simulink library "sm_wheel_loader_lib"  (R2025a)
settings: Solver=VariableStepAuto  StartTime=0.0  StopTime=10.0  RelTol=1e-3
undefined symbols (not defined in the file): AToTOrificeVector, BiPOrificeVector, boomHEArea, boomREArea, BToTOrificeVector, fluids, GRake, GToothL, GToothR, HMPST, HydFcnParams, logLoad, Position, PToAOrificeVector, PToBOrificeVector, RakeL, RakeR, testInput, Wheel_Loader, X, Y, Z
libraries: sm_lib x694, fl_lib x183, nesl_utility x74, SimscapeFluids_lib x62, sdl_lib x25, cvt_components_lib x25, simulink_extras x5, $bdroot x4, wheel_loader_contact_lib x4, ee_lib x2, SignalEditorBlockLib x1, batteryecm_lib x1
(part 5 of 26)

== system sm_wheel_loader_lib/CVT Power Split Hydromechanical/Hydrostatic/Motor Leakage ==
  Case Drain : fl_lib/Isothermal Liquid/Elements/Reservoir (IL)  reservoir_type=foundation.enum.constant_controlled.constant  pressure_spec=foundation.enum.pressure_spec.atmospheric  reservoir_pressure=0.101325 MPa
  Leakage A : fl_lib/Isothermal Liquid/Elements/Laminar Leakage (IL)  cross_section_geometry=foundation.enum.cross_section_geometry.custom  diameter=1e-3 m  inner_diameter=5e-4 m  outer_diameter=1e-3 m  width=1e-3 m  height=0.1 m  major_axis=1e-3 m  minor_axis=5e-4 m  side_length=1e-3 m  length=5 m  resistance=1e7 s*MPa/m^3
      settings: InternalSimscapePortConfiguration="{\"Bottom\":[],\"Left\":[{\"id\":\"A\",\"label\":\"A\",\"type\":\"foundation.isothermal_liquid.isothermal_liquid\"}],\"Right\":[{\"id\":\"B\",\"label\":\"B\",\"type\":\"foundation.isothermal_liquid.isothermal_liquid\"}],\"Top\":[]}"
  Leakage B : fl_lib/Isothermal Liquid/Elements/Laminar Leakage (IL)  cross_section_geometry=foundation.enum.cross_section_geometry.custom  diameter=1e-3 m  inner_diameter=5e-4 m  outer_diameter=1e-3 m  width=1e-3 m  height=0.1 m  major_axis=1e-3 m  minor_axis=5e-4 m  side_length=1e-3 m  length=5 m  resistance=1e7 s*MPa/m^3
      settings: InternalSimscapePortConfiguration="{\"Bottom\":[],\"Left\":[{\"id\":\"A\",\"label\":\"A\",\"type\":\"foundation.isothermal_liquid.isothermal_liquid\"}],\"Right\":[{\"id\":\"B\",\"label\":\"B\",\"type\":\"foundation.isothermal_liquid.isothermal_liquid\"}],\"Top\":[]}"
  A : PMIOPort  Side=Left
  B : PMIOPort  Port=2  Side=Left
  connections:
  Leakage A/LConn1 -- A/RConn1
  Leakage B/RConn1 -- Case Drain/LConn1 -- Leakage A/RConn1
  Leakage B/LConn1 -- B/RConn1

== system sm_wheel_loader_lib/CVT Power Split Hydromechanical/Hydrostatic/Pump Leakage ==
  Case Drain : fl_lib/Isothermal Liquid/Elements/Reservoir (IL)  reservoir_type=foundation.enum.constant_controlled.constant  pressure_spec=foundation.enum.pressure_spec.atmospheric  reservoir_pressure=0.101325 MPa
  Leakage A : fl_lib/Isothermal Liquid/Elements/Laminar Leakage (IL)  cross_section_geometry=foundation.enum.cross_section_geometry.custom  diameter=1e-3 m  inner_diameter=5e-4 m  outer_diameter=1e-3 m  width=1e-3 m  height=0.1 m  major_axis=1e-3 m  minor_axis=5e-4 m  side_length=1e-3 m  length=5 m  resistance=1e7 s*MPa/m^3
      settings: InternalSimscapePortConfiguration="{\"Bottom\":[],\"Left\":[{\"id\":\"A\",\"label\":\"A\",\"type\":\"foundation.isothermal_liquid.isothermal_liquid\"}],\"Right\":[{\"id\":\"B\",\"label\":\"B\",\"type\":\"foundation.isothermal_liquid.isothermal_liquid\"}],\"Top\":[]}"
  Leakage B : fl_lib/Isothermal Liquid/Elements/Laminar Leakage (IL)  cross_section_geometry=foundation.enum.cross_section_geometry.custom  diameter=1e-3 m  inner_diameter=5e-4 m  outer_diameter=1e-3 m  width=1e-3 m  height=0.1 m  major_axis=1e-3 m  minor_axis=5e-4 m  side_length=1e-3 m  length=5 m  resistance=1e7 s*MPa/m^3
      settings: InternalSimscapePortConfiguration="{\"Bottom\":[],\"Left\":[{\"id\":\"A\",\"label\":\"A\",\"type\":\"foundation.isothermal_liquid.isothermal_liquid\"}],\"Right\":[{\"id\":\"B\",\"label\":\"B\",\"type\":\"foundation.isothermal_liquid.isothermal_liquid\"}],\"Top\":[]}"
  B : PMIOPort  Side=Left
  A : PMIOPort  Port=2  Side=Left
  connections:
  Leakage A/LConn1 -- A/RConn1
  Leakage B/RConn1 -- Leakage A/RConn1 -- Case Drain/LConn1
  Leakage B/LConn1 -- B/RConn1

== system sm_wheel_loader_lib/Controller/CVT Ratio Ctrl/Range Calculation ==
  Ratio (-) : Inport
  Check Range 0 or higher : Switch  Threshold=XY_I(1,2)  SaturateOnIntegerOverflow=off  InputSameDT=off
  Check Range 2 or higher : Switch  Threshold=XY_I(2,2)  SaturateOnIntegerOverflow=off  InputSameDT=off
  Check Range 3 or higher : Switch  Threshold=XY_I(3,2)  SaturateOnIntegerOverflow=off  InputSameDT=off
  Check Range 4 : Switch  Threshold=XY_I(4,2)  SaturateOnIntegerOverflow=off  InputSameDT=off
  Constant1 : Constant  Value=2  SampleTime=HMPST.Simu.TimeStep
  Constant2 : Constant  SampleTime=HMPST.Simu.TimeStep
  Constant3 : Constant  Value=-1  SampleTime=HMPST.Simu.TimeStep
  Constant4 : Constant  Value=3  SampleTime=HMPST.Simu.TimeStep
  Constant5 : Constant  Value=4  SampleTime=HMPST.Simu.TimeStep
  Range (-) : Outport
  wires:
  Check Range 2 or higher/1 -> Check Range 0 or higher/1
  Constant2/1 -> Check Range 2 or higher/3
  Constant3/1 -> Check Range 0 or higher/3
  Check Range 0 or higher/1 -> Range (-)/1  "Range"
  Check Range 3 or higher/1 -> Check Range 2 or higher/1
  Constant1/1 -> Check Range 3 or higher/3
  Check Range 4/1 -> Check Range 3 or higher/1
  Constant4/1 -> Check Range 4/3
  Constant5/1 -> Check Range 4/1
  Ratio (-)/1 -> Check Range 2 or higher/2, Check Range 3 or higher/2, Check Range 4/2, Check Range 0 or higher/2

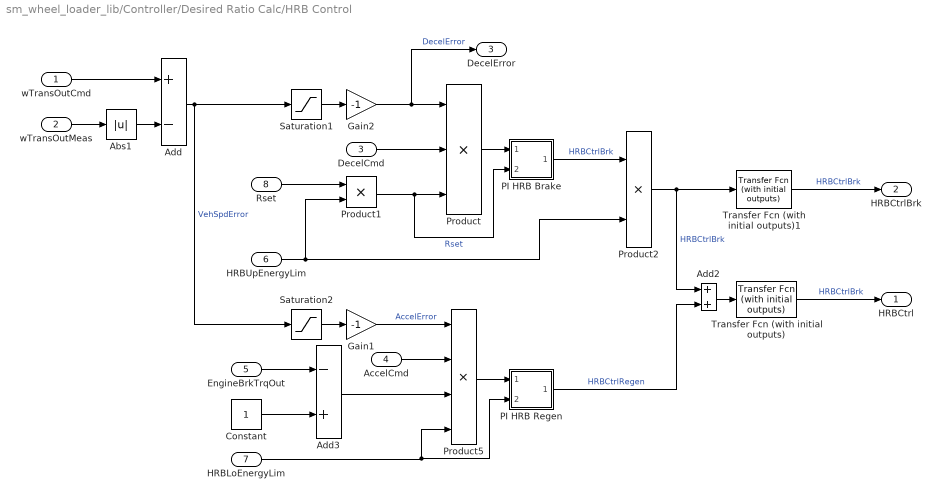
== system sm_wheel_loader_lib/Controller/Desired Ratio Calc/HRB Control ==
  wTransOutCmd : Inport
  wTransOutMeas : Inport  Port=2
  DecelCmd : Inport  Port=3
  AccelCmd : Inport  Port=4
  EngineBrkTrqOut : Inport  Port=5
  HRBUpEnergyLim : Inport  Port=6
  HRBLoEnergyLim : Inport  Port=7
  Rset : Inport  Port=8
  Abs1 : Abs  ZeroCross=off  SaturateOnIntegerOverflow=off
  Add : Sum  Inputs=+-
  Add2 : Sum
  Add3 : Sum  Inputs=-+
  Constant : Constant
  Gain1 : Gain  Gain=-1
  Gain2 : Gain  Gain=-1
  PI HRB Brake : Subsystem
  PI HRB Regen : Subsystem
  Product : Product  Inputs=3
  Product1 : Product
  Product2 : Product
  Product5 : Product  Inputs=4
  Saturation1 : Saturate  UpperLimit=0  LowerLimit=-inf  ZeroCross=off
  Saturation2 : Saturate  UpperLimit=inf  LowerLimit=0  ZeroCross=off
  Transfer Fcn (with initial outputs) : simulink_extras/Additional Linear/Transfer Fcn (with initial outputs)  N=[0.01]  D=[0.05 1]  Y0=0  U0=0
  Transfer Fcn (with initial outputs)1 : simulink_extras/Additional Linear/Transfer Fcn (with initial outputs)  N=[0.01]  D=[0.05 1]  Y0=0  U0=0
  HRBCtrl : Outport
  HRBCtrlBrk : Outport  Port=2
  DecelError : Outport  Port=3
  wires:
  Product/1 -> PI HRB Brake/1(error)
  Product5/1 -> PI HRB Regen/1(error)
  Gain1/1 -> Product5/1  "AccelError"
  Transfer Fcn (with initial outputs)1/1 -> HRBCtrlBrk/1  "HRBCtrlBrk"
  Rset/1 -> Product1/1
  EngineBrkTrqOut/1 -> Add3/1
  wTransOutCmd/1 -> Add/1
  PI HRB Brake/1(ctrl) -> Product2/1  "HRBCtrlBrk"
  wTransOutMeas/1 -> Abs1/1
  Gain2/1 -> Product/1, DecelError/1  "DecelError"
  AccelCmd/1 -> Product5/2
  Saturation1/1 -> Gain2/1
  Saturation2/1 -> Gain1/1
  PI HRB Regen/1(ctrl) -> Add2/2  "HRBCtrlRegen"
  HRBUpEnergyLim/1 -> Product1/2, Product2/2
  Abs1/1 -> Add/2
  DecelCmd/1 -> Product/2
  Product2/1 -> Transfer Fcn (with initial outputs)1/1, Add2/1  "HRBCtrlBrk"
  Add/1 -> Saturation1/1, Saturation2/1  "VehSpdError"
  Transfer Fcn (with initial outputs)/1 -> HRBCtrl/1  "HRBCtrlBrk"
  Constant/1 -> Add3/2
  Product1/1 -> Product/3, PI HRB Brake/2(Rset)  "Rset"
  Add3/1 -> Product5/3
  HRBLoEnergyLim/1 -> Product5/4, PI HRB Regen/2(Rset)
  Add2/1 -> Transfer Fcn (with initial outputs)/1

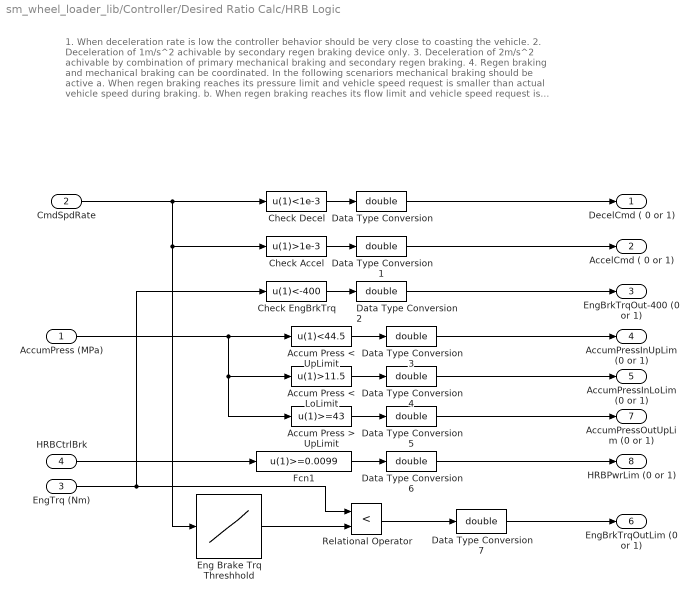
== system sm_wheel_loader_lib/Controller/Desired Ratio Calc/HRB Logic ==
  note: 1. When deceleration rate is low the controller behavior should be very close to coasting the vehicle.
      | 2. Deceleration of 1m/s^2 achivable by secondary regen braking device only.
      | 3. Deceleration of 2m/s^2 achivable by combination of primary mechanical braking and secondary regen braking.
      | 4. Regen braking and mechanical braking can be coordinated. In the following scenariors mechanical braking should be active
      | a. When regen braking reaches its pressure limit and vehicle speed request is smaller than actual vehicle speed during braking.
      | b. When regen braking reaches its flow limit and vehicle speed request is smaller than actual vehicle speed during braking.
      | 5. Energy in the accumulator will be released when accelerating and the accumulator pressure is above minimum working pressure.
      | Energy release rate should not cause engine over speeding.
      | 6. If engine over speed limit is reached disengage master clutch/shut down the engine.
  AccumPress (MPa) : Inport
  CmdSpdRate : Inport  Port=2
  EngTrq (Nm) : Inport  Port=3
  HRBCtrlBrk : Inport  Port=4
  Accum Press < LoLimit : Fcn  Expr=u(1)>11.5
  Accum Press < UpLimit : Fcn  Expr=u(1)<44.5
  Accum Press > UpLimit : Fcn  Expr=u(1)>=43
  Check Accel : Fcn  Expr=u(1)>1e-3
  Check Decel : Fcn  Expr=u(1)<1e-3
  Check EngBrkTrq : Fcn  Expr=u(1)<-400
  Data Type Conversion{,1..7} (8 alike) : DataTypeConversion  OutDataTypeStr=double  SaturateOnIntegerOverflow=off  RndMeth=Floor
  Eng Brake Trq Threshhold : Lookup_n-D  NumberOfTableDimensions=1  BreakpointsForDimension1=[-3 -2 -1 -0.5 0 1]  Table=[-450 -450 -225 -113 0 0]*0.6  InternalRulePriority=Speed  RndMeth=Simplest
  Fcn1 : Fcn  Expr=u(1)>=0.0099
  Relational Operator : RelationalOperator  Operator=<  OutDataTypeStr=boolean  ZeroCross=off  InputSameDT=off
  DecelCmd ( 0 or 1) : Outport
  AccelCmd ( 0 or 1) : Outport  Port=2
  EngBrkTrqOut-400 (0 or 1) : Outport  Port=3
  AccumPressInUpLim (0 or 1) : Outport  Port=4
  AccumPressInLoLim (0 or 1) : Outport  Port=5
  EngBrkTrqOutLim (0 or 1) : Outport  Port=6
  AccumPressOutUpLim (0 or 1) : Outport  Port=7
  HRBPwrLim (0 or 1) : Outport  Port=8
  wires:
  Check Decel/1 -> Data Type Conversion/1
  Data Type Conversion/1 -> DecelCmd ( 0 or 1)/1
  EngTrq (Nm)/1 -> Relational Operator/1, Check EngBrkTrq/1
  CmdSpdRate/1 -> Check Decel/1, Eng Brake Trq Threshhold/1, Check Accel/1
  Eng Brake Trq Threshhold/1 -> Relational Operator/2
  AccumPress (MPa)/1 -> Accum Press < LoLimit/1, Accum Press > UpLimit/1, Accum Press < UpLimit/1
  Accum Press < UpLimit/1 -> Data Type Conversion3/1
  Relational Operator/1 -> Data Type Conversion7/1
  Accum Press > UpLimit/1 -> Data Type Conversion5/1
  HRBCtrlBrk/1 -> Fcn1/1
  Fcn1/1 -> Data Type Conversion6/1
  Accum Press < LoLimit/1 -> Data Type Conversion4/1
  Check Accel/1 -> Data Type Conversion1/1
  Check EngBrkTrq/1 -> Data Type Conversion2/1
  Data Type Conversion1/1 -> AccelCmd ( 0 or 1)/1
  Data Type Conversion2/1 -> EngBrkTrqOut-400 (0 or 1)/1
  Data Type Conversion3/1 -> AccumPressInUpLim (0 or 1)/1
  Data Type Conversion4/1 -> AccumPressInLoLim (0 or 1)/1
  Data Type Conversion5/1 -> AccumPressOutUpLim (0 or 1)/1
  Data Type Conversion6/1 -> HRBPwrLim (0 or 1)/1
  Data Type Conversion7/1 -> EngBrkTrqOutLim (0 or 1)/1

== system sm_wheel_loader_lib/Controller/Desired Ratio Calc/MB Control ==
  Decel Error : Inport
  wTransOutCmd : Inport  Port=2
  Rset : Inport  Port=3
  AccumLimUp : Inport  Port=4
  HRBPowerLim : Inport  Port=5
  Add1 : Sum  Inputs=+++
  Compare To Constant : simulink/Logic and Bit Operations/Compare To Constant  relop=<=  const=0.02  OutDataTypeStr=boolean
  Data Type Conversion : DataTypeConversion  OutDataTypeStr=double  SaturateOnIntegerOverflow=off  RndMeth=Floor
  PI MB No HRB : Subsystem
  PI MB with MRB : Subsystem
  Product3 : Product  Inputs=3
  Product4 : Product
  Out1 : Outport
  wires:
  HRBPowerLim/1 -> Product4/2
  AccumLimUp/1 -> Product3/3
  wTransOutCmd/1 -> Compare To Constant/1
  PI MB with MRB/1(ctrl) -> Add1/3
  Add1/1 -> Out1/1
  Product4/1 -> PI MB with MRB/1(error)
  PI MB No HRB/1(ctrl) -> Add1/2
  Data Type Conversion/1 -> Add1/1
  Compare To Constant/1 -> Data Type Conversion/1
  Rset/1 -> PI MB with MRB/2(Rset), PI MB No HRB/2(Rset), Product3/2
  Product3/1 -> PI MB No HRB/1(error)
  Decel Error/1 -> Product4/1, Product3/1

== system sm_wheel_loader_lib/Controller/Desired Ratio Calc/VehSpdDir ==
  u : Inport
  Constant1 : Constant
  Constant2 : Constant  Value=-1
  Constant3 : Constant  Value=0
  Gain : Gain  Gain=-1
  Switch : Switch  Criteria=u2 > Threshold  Threshold=0.001  SaturateOnIntegerOverflow=off  InputSameDT=off
  Switch1 : Switch  Criteria=u2 > Threshold  Threshold=0.001  SaturateOnIntegerOverflow=off  InputSameDT=off
  u_dir : Outport
  wires:
  Gain/1 -> Switch1/2
  Switch/1 -> u_dir/1
  u/1 -> Switch/2, Gain/1
  Constant1/1 -> Switch/1
  Switch1/1 -> Switch/3
  Constant3/1 -> Switch1/3
  Constant2/1 -> Switch1/1

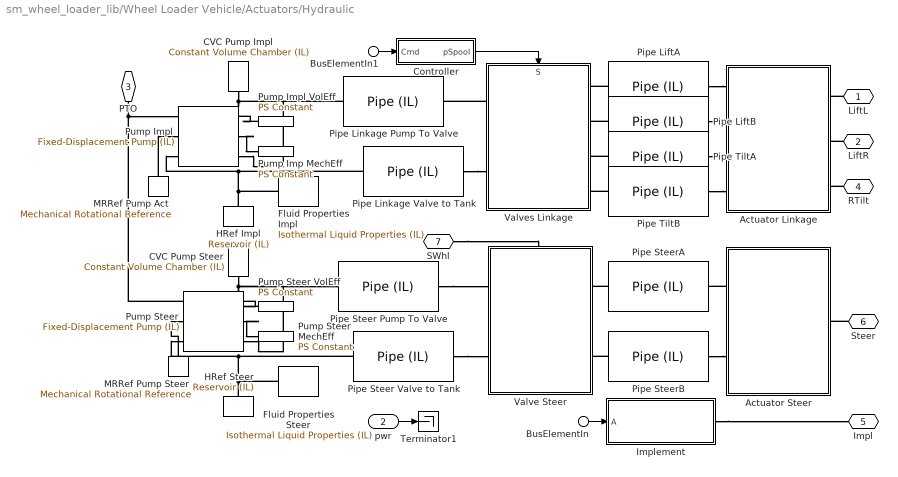
== system sm_wheel_loader_lib/Wheel Loader Vehicle/Actuators/Hydraulic ==
  BusElementIn : Inport  PortName=Cmd  Element=Actuator
  BusElementIn1 : Inport  PortName=Cmd  Element=Operator
  pwr : Inport  Port=2
  Actuator Linkage : Subsystem
      mask Display: image('sm_wheel_loader_actuator_linkage_IMAGE.png');
  Actuator Steer : Subsystem
      mask Display: image('sm_wheel_loader_actuator_steer_IMAGE.png');
  CVC Pump Impl : fl_lib/Isothermal Liquid/Elements/Constant Volume Chamber (IL)  volume=HydFcnParams.pump.chamberVol mm^3  p_I_specify=off  p_I_priority=High  p_I=0.101325 MPa  p_I_nominal_specify=off  p_I_nominal_value=1  p_I_nominal_unit=MPa
      settings: InternalSimscapePortConfiguration="{\"Bottom\":[],\"Left\":[{\"id\":\"A\",\"label\":\"A\",\"type\":\"foundation.isothermal_liquid.isothermal_liquid\"}],\"Right\":[],\"Top\":[]}"
  CVC Pump Steer : fl_lib/Isothermal Liquid/Elements/Constant Volume Chamber (IL)  volume=HydFcnParams.steerPump.chamberVol mm^3  p_I_specify=off  p_I_priority=High  p_I=0.101325 MPa  p_I_nominal_specify=off  p_I_nominal_value=1  p_I_nominal_unit=MPa
      settings: InternalSimscapePortConfiguration="{\"Bottom\":[],\"Left\":[{\"id\":\"A\",\"label\":\"A\",\"type\":\"foundation.isothermal_liquid.isothermal_liquid\"}],\"Right\":[],\"Top\":[]}"
  Controller : Subsystem
  Fluid Properties Impl : fl_lib/Isothermal Liquid/Utilities/Isothermal Liquid Properties (IL)  rho_L_atm=870 kg/m^3  bulk_modulus_model=foundation.enum.bulk_modulus_model.const  beta_gain=6  beta_L_atm=1.45e9 Pa  nu_atm=46 mm^2/s  p_atm=0.101325 MPa  p_min=0.1 Pa  properties_range_check=simscape.enum.assert.action.error  air_fraction=0.005  polytropic_index=1.0  rho_g_atm=1.225 kg/m^3  air_dissolution_model=simscape.enum.onoff.off  p_crit=3 MPa
  Fluid Properties Steer : fl_lib/Isothermal Liquid/Utilities/Isothermal Liquid Properties (IL)  rho_L_atm=870 kg/m^3  bulk_modulus_model=foundation.enum.bulk_modulus_model.const  beta_gain=6  beta_L_atm=1.45e9 Pa  nu_atm=46 mm^2/s  p_atm=0.101325 MPa  p_min=0.1 Pa  properties_range_check=simscape.enum.assert.action.error  air_fraction=0.005  polytropic_index=1.0  rho_g_atm=1.225 kg/m^3  air_dissolution_model=simscape.enum.onoff.off  p_crit=3 MPa
  HRef Impl : fl_lib/Isothermal Liquid/Elements/Reservoir (IL)  reservoir_type=foundation.enum.constant_controlled.constant  pressure_spec=foundation.enum.pressure_spec.atmospheric  reservoir_pressure=0.101325 MPa
  HRef Steer : fl_lib/Isothermal Liquid/Elements/Reservoir (IL)  reservoir_type=foundation.enum.constant_controlled.constant  pressure_spec=foundation.enum.pressure_spec.atmospheric  reservoir_pressure=0.101325 MPa
  Implement : Subsystem  Variant=on  VariantControlMode=label  VariantControl=Grapple Rake  LabelModeActiveChoice=Bucket
      settings: AttributesFormatString=%<LabelModeActiveChoice>
  MRRef Pump Act : fl_lib/Mechanical/Rotational Elements/Mechanical Rotational Reference
  MRRef Pump Steer : fl_lib/Mechanical/Rotational Elements/Mechanical Rotational Reference
  Pipe LiftA : fl_lib/Isothermal Liquid/Elements/Pipe (IL)  length=HydFcnParams.pipes.length mm  area=HydFcnParams.pipe.crossSectArea mm^2  Dh=HydFcnParams.pipes.hydraulicDiam mm  length_add=1 m  roughness=15e-6 m  Re_lam=2000  Re_tur=4000  shape_factor=64  dynamic_compressibility=simscape.enum.onoff.off  inertia=simscape.enum.onoff.off  p0=0.101325 MPa  mdot0=0 kg/s
      settings: InternalSimscapePortConfiguration="{\"Bottom\":[],\"Left\":[{\"id\":\"A\",\"label\":\"A\",\"type\":\"foundation.isothermal_liquid.isothermal_liquid\"}],\"Right\":[{\"id\":\"B\",\"label\":\"B\",\"type\":\"foundation.isothermal_liquid.isothermal_liquid\"}],\"Top\":[]}"
  Pipe LiftB : fl_lib/Isothermal Liquid/Elements/Pipe (IL)  length=HydFcnParams.pipes.length mm  area=HydFcnParams.pipe.crossSectArea mm^2  Dh=HydFcnParams.pipes.hydraulicDiam mm  length_add=1 m  roughness=15e-6 m  Re_lam=2000  Re_tur=4000  shape_factor=64  dynamic_compressibility=simscape.enum.onoff.off  inertia=simscape.enum.onoff.off  p0=0.101325 MPa  mdot0=0 kg/s
      settings: InternalSimscapePortConfiguration="{\"Bottom\":[],\"Left\":[{\"id\":\"A\",\"label\":\"A\",\"type\":\"foundation.isothermal_liquid.isothermal_liquid\"}],\"Right\":[{\"id\":\"B\",\"label\":\"B\",\"type\":\"foundation.isothermal_liquid.isothermal_liquid\"}],\"Top\":[]}"
  Pipe Linkage Pump To Valve : fl_lib/Isothermal Liquid/Elements/Pipe (IL)  length=HydFcnParams.pipes.length mm  area=HydFcnParams.pipe.crossSectArea mm^2  Dh=HydFcnParams.pipes.hydraulicDiam mm  length_add=1 m  roughness=15e-6 m  Re_lam=2000  Re_tur=4000  shape_factor=64  dynamic_compressibility=simscape.enum.onoff.off  inertia=simscape.enum.onoff.off  p0=0.101325 MPa  mdot0=0 kg/s
      settings: InternalSimscapePortConfiguration="{\"Bottom\":[],\"Left\":[{\"id\":\"A\",\"label\":\"A\",\"type\":\"foundation.isothermal_liquid.isothermal_liquid\"}],\"Right\":[{\"id\":\"B\",\"label\":\"B\",\"type\":\"foundation.isothermal_liquid.isothermal_liquid\"}],\"Top\":[]}"
  Pipe Linkage Valve to Tank : fl_lib/Isothermal Liquid/Elements/Pipe (IL)  length=HydFcnParams.pipes.length mm  area=HydFcnParams.pipe.crossSectArea mm^2  Dh=HydFcnParams.pipes.hydraulicDiam mm  length_add=1 m  roughness=15e-6 m  Re_lam=2000  Re_tur=4000  shape_factor=64  dynamic_compressibility=simscape.enum.onoff.off  inertia=simscape.enum.onoff.off  p0=0.101325 MPa  mdot0=0 kg/s
      settings: InternalSimscapePortConfiguration="{\"Bottom\":[],\"Left\":[{\"id\":\"A\",\"label\":\"A\",\"type\":\"foundation.isothermal_liquid.isothermal_liquid\"}],\"Right\":[{\"id\":\"B\",\"label\":\"B\",\"type\":\"foundation.isothermal_liquid.isothermal_liquid\"}],\"Top\":[]}"
  Pipe Steer Pump To Valve : fl_lib/Isothermal Liquid/Elements/Pipe (IL)  length=HydFcnParams.pipes.length mm  area=HydFcnParams.pipe.crossSectArea mm^2  Dh=HydFcnParams.pipes.hydraulicDiam mm  length_add=1 m  roughness=15e-6 m  Re_lam=2000  Re_tur=4000  shape_factor=64  dynamic_compressibility=simscape.enum.onoff.off  inertia=simscape.enum.onoff.off  p0=0.101325 MPa  mdot0=0 kg/s
      settings: InternalSimscapePortConfiguration="{\"Bottom\":[],\"Left\":[{\"id\":\"A\",\"label\":\"A\",\"type\":\"foundation.isothermal_liquid.isothermal_liquid\"}],\"Right\":[{\"id\":\"B\",\"label\":\"B\",\"type\":\"foundation.isothermal_liquid.isothermal_liquid\"}],\"Top\":[]}"
  Pipe Steer Valve to Tank : fl_lib/Isothermal Liquid/Elements/Pipe (IL)  length=HydFcnParams.pipes.length mm  area=HydFcnParams.pipe.crossSectArea mm^2  Dh=HydFcnParams.pipes.hydraulicDiam mm  length_add=1 m  roughness=15e-6 m  Re_lam=2000  Re_tur=4000  shape_factor=64  dynamic_compressibility=simscape.enum.onoff.off  inertia=simscape.enum.onoff.off  p0=0.101325 MPa  mdot0=0 kg/s
      settings: InternalSimscapePortConfiguration="{\"Bottom\":[],\"Left\":[{\"id\":\"A\",\"label\":\"A\",\"type\":\"foundation.isothermal_liquid.isothermal_liquid\"}],\"Right\":[{\"id\":\"B\",\"label\":\"B\",\"type\":\"foundation.isothermal_liquid.isothermal_liquid\"}],\"Top\":[]}"
  Pipe SteerA : fl_lib/Isothermal Liquid/Elements/Pipe (IL)  length=HydFcnParams.pipes.length mm  area=HydFcnParams.pipe.crossSectArea mm^2  Dh=HydFcnParams.pipes.hydraulicDiam mm  length_add=1 m  roughness=15e-6 m  Re_lam=2000  Re_tur=4000  shape_factor=64  dynamic_compressibility=simscape.enum.onoff.off  inertia=simscape.enum.onoff.off  p0=0.101325 MPa  mdot0=0 kg/s
      settings: InternalSimscapePortConfiguration="{\"Bottom\":[],\"Left\":[{\"id\":\"A\",\"label\":\"A\",\"type\":\"foundation.isothermal_liquid.isothermal_liquid\"}],\"Right\":[{\"id\":\"B\",\"label\":\"B\",\"type\":\"foundation.isothermal_liquid.isothermal_liquid\"}],\"Top\":[]}"
  Pipe SteerB : fl_lib/Isothermal Liquid/Elements/Pipe (IL)  length=HydFcnParams.pipes.length mm  area=HydFcnParams.pipe.crossSectArea mm^2  Dh=HydFcnParams.pipes.hydraulicDiam mm  length_add=1 m  roughness=15e-6 m  Re_lam=2000  Re_tur=4000  shape_factor=64  dynamic_compressibility=simscape.enum.onoff.off  inertia=simscape.enum.onoff.off  p0=0.101325 MPa  mdot0=0 kg/s
      settings: InternalSimscapePortConfiguration="{\"Bottom\":[],\"Left\":[{\"id\":\"A\",\"label\":\"A\",\"type\":\"foundation.isothermal_liquid.isothermal_liquid\"}],\"Right\":[{\"id\":\"B\",\"label\":\"B\",\"type\":\"foundation.isothermal_liquid.isothermal_liquid\"}],\"Top\":[]}"
  Pipe TiltA : fl_lib/Isothermal Liquid/Elements/Pipe (IL)  length=HydFcnParams.pipes.length mm  area=HydFcnParams.pipe.crossSectArea mm^2  Dh=HydFcnParams.pipes.hydraulicDiam mm  length_add=1 m  roughness=15e-6 m  Re_lam=2000  Re_tur=4000  shape_factor=64  dynamic_compressibility=simscape.enum.onoff.off  inertia=simscape.enum.onoff.off  p0=0.101325 MPa  mdot0=0 kg/s
      settings: InternalSimscapePortConfiguration="{\"Bottom\":[],\"Left\":[{\"id\":\"A\",\"label\":\"A\",\"type\":\"foundation.isothermal_liquid.isothermal_liquid\"}],\"Right\":[{\"id\":\"B\",\"label\":\"B\",\"type\":\"foundation.isothermal_liquid.isothermal_liquid\"}],\"Top\":[]}"
  Pipe TiltB : fl_lib/Isothermal Liquid/Elements/Pipe (IL)  length=HydFcnParams.pipes.length mm  area=HydFcnParams.pipe.crossSectArea mm^2  Dh=HydFcnParams.pipes.hydraulicDiam mm  length_add=1 m  roughness=15e-6 m  Re_lam=2000  Re_tur=4000  shape_factor=64  dynamic_compressibility=simscape.enum.onoff.off  inertia=simscape.enum.onoff.off  p0=0.101325 MPa  mdot0=0 kg/s
      settings: InternalSimscapePortConfiguration="{\"Bottom\":[],\"Left\":[{\"id\":\"A\",\"label\":\"A\",\"type\":\"foundation.isothermal_liquid.isothermal_liquid\"}],\"Right\":[{\"id\":\"B\",\"label\":\"B\",\"type\":\"foundation.isothermal_liquid.isothermal_liquid\"}],\"Top\":[]}"
  Pump Impl : SimscapeFluids_lib/Isothermal Liquid/Pumps & Motors/Fixed-Displacement Pump (IL)  leakage_friction_spec=fluids.isothermal_liquid.pumps_motors.enum.pump_motor_loss_spec.input_efficiency  displacement=HydFcnParams.pump.displacement cm^3/rev  omega_nominal=HydFcnParams.pump.nomSpeed rpm  p_nominal=HydFcnParams.pump.nomPrGain bar  vol_eff_nominal=HydFcnParams.pump.volEff  mech_eff_nominal=HydFcnParams.pump.mechEff  no_load_torque=0 N*m  p_diff_eff_TLU=[.1, 1, 2] MPa  omega_eff_TLU=[250, 500, 1000, 2000, 3000, 4000] rpm  vol_eff_TLU=[.816, .908, .954, .977, .981, .984; .325, .663, .831, .916, .925, .946; .137, .568, .78, .892, .893, .91]  mech_eff_TLU=[.996, .996, .996, .996, .996, .996; .988, .989, .989, .989, .989, .99; .981, .981, .982, .982, .983, .984]  p_diff_loss_TLU=[.1, 1, 2] MPa  omega_loss_TLU=[250, 500, 1000, 2000, 3000, 4000] rpm  vol_loss_TLU=1e-3 * [.023, .023, .023, .023, .0285, .032; .0844, .0842, .0845, .084, .1125, .108; .1079, .108, .11, .108, .1605, .18] m^3/s  mech_loss_TLU=[.002, .002, .002, .002, .002, .002; .0607, .0556, .0556, .0556, .0556, .0505; .1937, .1937, .1833, .1833, .1729, .1626] N*m  vol_eff_min=1e-3  vol_eff_max=1  mech_eff_min=1e-3  mech_eff_max=1  pressure_threshold=1e-3 MPa  omega_threshold=100 rpm  supplied_range_check=simscape.enum.assert.action.none  pump_mode_check=simscape.enum.assert.action.none  pressure_check=simscape.enum.assert.action.none  p_min_valid=0.101325 MPa
      settings: InternalSimscapePortConfiguration="{\"Bottom\":[{\"id\":\"A\",\"label\":\"A\",\"type\":\"foundation.isothermal_liquid.isothermal_liquid\"}],\"Left\":[{\"id\":\"EV\",\"label\":\"EV\",\"type\":\"input\"},{\"id\":\"EM\",\"label\":\"EM\",\"type\":\"input\"}],\"Right\":[{\"id\":\"R\",\"label\":\"R\",\"type\":\"foundation.mechanical.rotational.rotational\"},{\"id\":\"C\",\"label\":\"C\",\"type\":\"foundation.mechanical.rotational.rotational\"}],\"Top\":[{\"id\":\"B\",\"label\":\"B\",\"type\":\"foundation.isothermal_liquid.isothermal_liquid\"}]}"
  Pump Steer : SimscapeFluids_lib/Isothermal Liquid/Pumps & Motors/Fixed-Displacement Pump (IL)  leakage_friction_spec=fluids.isothermal_liquid.pumps_motors.enum.pump_motor_loss_spec.input_efficiency  displacement=HydFcnParams.steerPump.displacement cm^3/rev  omega_nominal=HydFcnParams.pump.nomSpeed rpm  p_nominal=HydFcnParams.pump.nomPrGain bar  vol_eff_nominal=HydFcnParams.pump.volEff  mech_eff_nominal=HydFcnParams.pump.mechEff  no_load_torque=0 N*m  p_diff_eff_TLU=[.1, 1, 2] MPa  omega_eff_TLU=[250, 500, 1000, 2000, 3000, 4000] rpm  vol_eff_TLU=[.816, .908, .954, .977, .981, .984; .325, .663, .831, .916, .925, .946; .137, .568, .78, .892, .893, .91]  mech_eff_TLU=[.996, .996, .996, .996, .996, .996; .988, .989, .989, .989, .989, .99; .981, .981, .982, .982, .983, .984]  p_diff_loss_TLU=[.1, 1, 2] MPa  omega_loss_TLU=[250, 500, 1000, 2000, 3000, 4000] rpm  vol_loss_TLU=1e-3 * [.023, .023, .023, .023, .0285, .032; .0844, .0842, .0845, .084, .1125, .108; .1079, .108, .11, .108, .1605, .18] m^3/s  mech_loss_TLU=[.002, .002, .002, .002, .002, .002; .0607, .0556, .0556, .0556, .0556, .0505; .1937, .1937, .1833, .1833, .1729, .1626] N*m  vol_eff_min=1e-3  vol_eff_max=1  mech_eff_min=1e-3  mech_eff_max=1  pressure_threshold=1e-3 MPa  omega_threshold=100 rpm  supplied_range_check=simscape.enum.assert.action.none  pump_mode_check=simscape.enum.assert.action.none  pressure_check=simscape.enum.assert.action.none  p_min_valid=0.101325 MPa
      settings: InternalSimscapePortConfiguration="{\"Bottom\":[{\"id\":\"A\",\"label\":\"A\",\"type\":\"foundation.isothermal_liquid.isothermal_liquid\"}],\"Left\":[{\"id\":\"EV\",\"label\":\"EV\",\"type\":\"input\"},{\"id\":\"EM\",\"label\":\"EM\",\"type\":\"input\"}],\"Right\":[{\"id\":\"R\",\"label\":\"R\",\"type\":\"foundation.mechanical.rotational.rotational\"},{\"id\":\"C\",\"label\":\"C\",\"type\":\"foundation.mechanical.rotational.rotational\"}],\"Top\":[{\"id\":\"B\",\"label\":\"B\",\"type\":\"foundation.isothermal_liquid.isothermal_liquid\"}]}"
  Pump Imp MechEff : fl_lib/Physical Signals/Sources/PS Constant  constant=HydFcnParams.pump.mechEff
  Pump Impl VolEff : fl_lib/Physical Signals/Sources/PS Constant  constant=HydFcnParams.pump.volEff
  Pump Steer MechEff : fl_lib/Physical Signals/Sources/PS Constant  constant=HydFcnParams.steerPump.mechEff
  Pump Steer VolEff : fl_lib/Physical Signals/Sources/PS Constant  constant=HydFcnParams.steerPump.volEff
  Terminator1 : Terminator
  Valve Steer : Subsystem
      settings: PortSchema="{\"entries\":[{\"content\":{\"sides\":[{\"content\":{\"connectorIds\":[\"LConn1\",\"LConn2\"]},\"type\":\"ConnectorPlacement.EquallySpacedRectSide\",\"uuid\":\"408e1035-6b3d-4519-b3f1-e009707ee901\"},{\"content\":{\"connectorIds\":[\"RConn1\",\"RConn2\"],\"side\":\"RIGHT\"},\"type\":\"ConnectorPlacement.EquallySpacedRectSide\",\"uuid\":\"f6fc5ec3-963d-4896-a810-4c1d83a284ca\"},{\"content\":{\"connectorIds\":[\"LConn3\"],\"side\":\"TOP\"},\"type\":\"ConnectorPlacement.EquallySpacedRectSide\",\"uuid\":\"5ee59ebc-e402-4785-9120-6ae47dd60b43\"},{\"content\":{\"side\":\"BOTTOM\"},\"type\":\"ConnectorPlacement.EquallySpacedRectSide\",\"uuid\":\"a994d606-c935-4c5d-b566-9fce03890d2a\"}]},\"type\":\"ConnectorPlacement.EquallySpacedConnector\",\"uuid\":\"c6791463-b308-429c-8dd1-d15f50199213\"}],\"packageUris\":[\"http://schema.mathworks.com/mf0/Connector/R2020b\"],\"version\":\"1.0\"}"
      mask Display: image('sm_wheel_loader_valve_gerotor_IMAGE.png');
  Valves Linkage : Subsystem
      settings: PortSchema="{\"entries\":[{\"content\":{\"sides\":[{\"content\":{\"connectorIds\":[\"LConn1\",\"LConn2\"]},\"type\":\"ConnectorPlacement.EquallySpacedRectSide\",\"uuid\":\"e97bc73b-9f55-4fad-8581-2066e0d00398\"},{\"content\":{\"connectorIds\":[\"RConn1\",\"RConn2\",\"RConn3\",\"RConn4\"],\"side\":\"RIGHT\"},\"type\":\"ConnectorPlacement.EquallySpacedRectSide\",\"uuid\":\"96a7ce6b-69e5-4ab0-8b6a-18f7c232fee9\"},{\"content\":{\"connectorIds\":[\"In1\"],\"side\":\"TOP\"},\"type\":\"ConnectorPlacement.EquallySpacedRectSide\",\"uuid\":\"ae84efc8-1053-4ca4-8a9f-7b6269b642b7\"}]},\"type\":\"ConnectorPlacement.EquallySpacedConnector\",\"uuid\":\"dc6a267f-cf26-460c-b9d1-1342509ba07b\"}],\"packageUris\":[\"http://schema.mathworks.com/mf0/Connector/R2020b\"],\"version\":\"1.0\"}"
      mask Display: image('sm_wheel_loader_valve_linkage_IMAGE.png');
  LiftL : PMIOPort  Side=Right
  LiftR : PMIOPort  Port=2  Side=Right
  PTO : PMIOPort  Port=3  Side=Left
  RTilt : PMIOPort  Port=4  Side=Left
  Impl : PMIOPort  Port=5  Side=Right
  Steer : PMIOPort  Port=6  Side=Right
  SWhl : PMIOPort  Port=7  Side=Left
  wires:
  BusElementIn1/1 -> Controller/1(Cmd)
  BusElementIn/1 -> Implement/1(A)
  Controller/1(pSpool) -> Valves Linkage/1(S)
  pwr/1 -> Terminator1/1
  connections:
  Pump Steer/RConn1 -- Pump Impl/RConn1 -- PTO/RConn1
  Implement/RConn1 -- Impl/RConn1
  Steer/RConn1 -- Actuator Steer/RConn1
  LiftR/RConn1 -- Actuator Linkage/RConn2
  MRRef Pump Steer/LConn1 -- Pump Steer/RConn2
  MRRef Pump Act/LConn1 -- Pump Impl/RConn2
  Pipe Steer Pump To Valve/RConn1 -- Valve Steer/LConn1
  Pump Steer/LConn2 -- Pump Steer MechEff/RConn1
  Pump Steer VolEff/RConn1 -- Pump Steer/LConn1
  Pipe Steer Valve to Tank/LConn1 -- Valve Steer/LConn2
  CVC Pump Steer/LConn1 -- Pump Steer/LConn3 -- Pipe Steer Pump To Valve/LConn1
  Fluid Properties Steer/RConn1 -- Pipe Steer Valve to Tank/RConn1 -- Pump Steer/RConn3 -- HRef Steer/LConn1
  Pipe SteerB/LConn1 -- Valve Steer/RConn2
  Pipe SteerA/LConn1 -- Valve Steer/RConn1
  RTilt/RConn1 -- Actuator Linkage/RConn3
  Actuator Steer/LConn1 -- Pipe SteerA/RConn1
  Pipe SteerB/RConn1 -- Actuator Steer/LConn2
  Pipe TiltB/RConn1 -- Actuator Linkage/LConn4
  Pipe TiltA/RConn1 -- Actuator Linkage/LConn3
  Pipe LiftB/RConn1 -- Actuator Linkage/LConn2
  Pipe LiftA/RConn1 -- Actuator Linkage/LConn1
  LiftL/RConn1 -- Actuator Linkage/RConn1
  Pipe TiltB/LConn1 -- Valves Linkage/RConn4
  Pipe TiltA/LConn1 -- Valves Linkage/RConn3
  Pipe LiftB/LConn1 -- Valves Linkage/RConn2
  Pipe LiftA/LConn1 -- Valves Linkage/RConn1
  Pipe Linkage Valve to Tank/LConn1 -- Valves Linkage/LConn2
  Valves Linkage/LConn1 -- Pipe Linkage Pump To Valve/RConn1
  HRef Impl/LConn1 -- Pipe Linkage Valve to Tank/RConn1 -- Pump Impl/RConn3 -- Fluid Properties Impl/RConn1
  Pipe Linkage Pump To Valve/LConn1 -- Pump Impl/LConn3 -- CVC Pump Impl/LConn1
  Pump Impl/LConn2 -- Pump Imp MechEff/RConn1
  Pump Impl VolEff/RConn1 -- Pump Impl/LConn1
  SWhl/RConn1 -- Valve Steer/LConn3

== system sm_wheel_loader_lib/Wheel Loader Vehicle/Actuators/Ideal ==
  note: The actuation of the cylinders is done through prescribed motion at the joints.
  Cmd : Inport
  pwr : Inport  Port=2
  Power Draw : Subsystem
  Shaft Inertia : fl_lib/Mechanical/Rotational Elements/Inertia  inertia=0.01 kg*m^2  num_ports=foundation.enum.numPorts2.one  w_specify=on  w_priority=None  w=0 rad/s  w_nominal_specify=off  w_nominal_value=1  w_nominal_unit=rad/s  t_specify=off  t_priority=None  t=0 N*m  t_nominal_specify=off  t_nominal_value=1  t_nominal_unit=N*m
  Steering Mechanism Inertia : fl_lib/Mechanical/Rotational Elements/Inertia  inertia=0.01 kg*m^2  num_ports=foundation.enum.numPorts2.one  w_specify=off  w_priority=High  w=0 rad/s  w_nominal_specify=off  w_nominal_value=1  w_nominal_unit=rad/s  t_specify=off  t_priority=None  t=0 N*m  t_nominal_specify=off  t_nominal_value=1  t_nominal_unit=N*m
  Terminator : Terminator
  LiftL : PMIOPort  Side=Right
  LiftR : PMIOPort  Port=2  Side=Right
  PTO : PMIOPort  Port=3  Side=Left
  RTilt : PMIOPort  Port=4  Side=Left
  Impl : PMIOPort  Port=5  Side=Right
  Steer : PMIOPort  Port=6  Side=Right
  SWhl : PMIOPort  Port=7  Side=Left
  wires:
  Cmd/1 -> Terminator/1
  pwr/1 -> Power Draw/1(pwr)
  connections:
  PTO/RConn1 -- Power Draw/RConn1 -- Shaft Inertia/LConn1
  Steering Mechanism Inertia/LConn1 -- SWhl/RConn1

== system sm_wheel_loader_lib/Wheel Loader Vehicle/Driveline/Axle Housing Front ==
  Bearing : sm_lib/Body Elements/File Solid  ExtGeomFileName=AxleF_Housing_Bearing.STEP  UnitType=FromFile  ExtGeomFileUnits=m  StepReaderType=HEX  ExportConvexHullGeometry=off  InertiaType=Custom  BasedOnType=DensityFromFile  Density=1000  DensityUnits=kg/m^3  Mass=Wheel_Loader.bodyGroups(36).subGroups(2).inertialProperties.mass  MassUnits=kg  CenterOfMass=Wheel_Loader.bodyGroups(36).subGroups(2).inertialProperties.centerOfMass  CenterOfMassUnits=m  MomentsOfInertia=Wheel_Loader.bodyGroups(36).subGroups(2).inertialProperties.momentsOfInertia  MomentsOfInertiaUnits=kg*m^2  ProductsOfInertia=Wheel_Loader.bodyGroups(36).subGroups(2).inertialProperties.productsOfInertia  ProductsOfInertiaUnits=kg*m^2  GraphicType=FromGeometry  MarkerShape=Sphere  MarkerSize=10  GraphicVisPropType=SimpleVisualProperties  GraphicDiffuseColor=Wheel_Loader.bodyGroups(36).subGroups(2).visualProperties.rgb  GraphicOpacity=fa_casing_opc  GraphicSpecularColor=[0.5 0.5 0.5 1.0]  GraphicAmbientColor=[0.15 0.15 0.15 1.0]  GraphicEmissiveColor=[0.0 0.0 0.0 1.0]  GraphicShininess=75  DoExposeReferenceFrame=on  SerializedFrames=<Frames/>
  Bolts : sm_lib/Body Elements/File Solid  ExtGeomFileName=AxleF_Housing_Bolts.STEP  UnitType=FromFile  ExtGeomFileUnits=m  StepReaderType=HEX  ExportConvexHullGeometry=off  InertiaType=Custom  BasedOnType=DensityFromFile  Density=1000  DensityUnits=kg/m^3  Mass=Wheel_Loader.bodyGroups(36).subGroups(3).inertialProperties.mass  MassUnits=kg  CenterOfMass=Wheel_Loader.bodyGroups(36).subGroups(3).inertialProperties.centerOfMass  CenterOfMassUnits=m  MomentsOfInertia=Wheel_Loader.bodyGroups(36).subGroups(3).inertialProperties.momentsOfInertia  MomentsOfInertiaUnits=kg*m^2  ProductsOfInertia=Wheel_Loader.bodyGroups(36).subGroups(3).inertialProperties.productsOfInertia  ProductsOfInertiaUnits=kg*m^2  GraphicType=FromGeometry  MarkerShape=Sphere  MarkerSize=10  GraphicVisPropType=SimpleVisualProperties  GraphicDiffuseColor=Wheel_Loader.bodyGroups(36).subGroups(3).visualProperties.rgb  GraphicOpacity=fa_casing_opc  GraphicSpecularColor=[0.5 0.5 0.5 1.0]  GraphicAmbientColor=[0.15 0.15 0.15 1.0]  GraphicEmissiveColor=[0.0 0.0 0.0 1.0]  GraphicShininess=75  DoExposeReferenceFrame=on  SerializedFrames=<Frames/>
  Housing : sm_lib/Body Elements/File Solid  ExtGeomFileName=AxleF_Housing.STEP  UnitType=FromFile  ExtGeomFileUnits=m  StepReaderType=HEX  ExportConvexHullGeometry=off  InertiaType=Custom  BasedOnType=DensityFromFile  Density=1000  DensityUnits=kg/m^3  Mass=Wheel_Loader.bodyGroups(36).subGroups(1).inertialProperties.mass  MassUnits=kg  CenterOfMass=Wheel_Loader.bodyGroups(36).subGroups(1).inertialProperties.centerOfMass  CenterOfMassUnits=m  MomentsOfInertia=Wheel_Loader.bodyGroups(36).subGroups(1).inertialProperties.momentsOfInertia  MomentsOfInertiaUnits=kg*m^2  ProductsOfInertia=Wheel_Loader.bodyGroups(36).subGroups(1).inertialProperties.productsOfInertia  ProductsOfInertiaUnits=kg*m^2  GraphicType=FromGeometry  MarkerShape=Sphere  MarkerSize=10  GraphicVisPropType=SimpleVisualProperties  GraphicDiffuseColor=Wheel_Loader.bodyGroups(36).subGroups(1).visualProperties.rgb  GraphicOpacity=fa_casing_opc  GraphicSpecularColor=[0.5 0.5 0.5 1.0]  GraphicAmbientColor=[0.15 0.15 0.15 1.0]  GraphicEmissiveColor=[0.0 0.0 0.0 1.0]  GraphicShininess=75  DoExposeReferenceFrame=on  SerializedFrames=<Frames/>
  RT_FrontAxle_FDPinion : sm_lib/Frames and Transforms/Rigid Transform  RotationMethod=RotationMatrix  FollAlignAxisA=+X  BaseAlignAxisA=+Y  FollAlignAxisB=+Y  BaseAlignAxisB=+Z  RotationStandardAxis=+Z  RotationAngle=0.0  RotationAngleUnits=deg  RotationArbitraryAxis=[0 0 1]  RotationSequenceAxes=FollowerAxes  RotationSequence=XYX  RotationSequenceAngles=[0 0 0]  RotationSequenceAnglesUnits=deg  RotationMatrix=Wheel_Loader.coordSys(44).transform.rotation  Quaternion=[1 0 0 0]  TranslationMethod=Cartesian  TranslationCartesianOffset=Wheel_Loader.coordSys(44).transform.translation  TranslationCartesianOffsetUnits=m  TranslationStandardAxis=+Z  TranslationStandardOffset=0  TranslationStandardOffsetUnits=m  TranslationROffset=0  TranslationROffsetUnits=m  TranslationThetaOffset=0  TranslationThetaOffsetUnits=deg  TranslationZOffset=0  TranslationZOffsetUnits=m
  RT_FrontAxle_LFFDRing_Weld : sm_lib/Frames and Transforms/Rigid Transform  RotationMethod=RotationMatrix  FollAlignAxisA=+X  BaseAlignAxisA=+Y  FollAlignAxisB=+Y  BaseAlignAxisB=+Z  RotationStandardAxis=+Z  RotationAngle=0.0  RotationAngleUnits=deg  RotationArbitraryAxis=[0 0 1]  RotationSequenceAxes=FollowerAxes  RotationSequence=XYX  RotationSequenceAngles=[0 0 0]  RotationSequenceAnglesUnits=deg  RotationMatrix=Wheel_Loader.coordSys(70).transform.rotation  Quaternion=[1 0 0 0]  TranslationMethod=Cartesian  TranslationCartesianOffset=Wheel_Loader.coordSys(70).transform.translation  TranslationCartesianOffsetUnits=m  TranslationStandardAxis=+Z  TranslationStandardOffset=0  TranslationStandardOffsetUnits=m  TranslationROffset=0  TranslationROffsetUnits=m  TranslationThetaOffset=0  TranslationThetaOffsetUnits=deg  TranslationZOffset=0  TranslationZOffsetUnits=m
  RT_FrontAxle_RFFDRing_Weld : sm_lib/Frames and Transforms/Rigid Transform  RotationMethod=RotationMatrix  FollAlignAxisA=+X  BaseAlignAxisA=+Y  FollAlignAxisB=+Y  BaseAlignAxisB=+Z  RotationStandardAxis=+Z  RotationAngle=0.0  RotationAngleUnits=deg  RotationArbitraryAxis=[0 0 1]  RotationSequenceAxes=FollowerAxes  RotationSequence=XYX  RotationSequenceAngles=[0 0 0]  RotationSequenceAnglesUnits=deg  RotationMatrix=Wheel_Loader.coordSys(66).transform.rotation  Quaternion=[1 0 0 0]  TranslationMethod=Cartesian  TranslationCartesianOffset=Wheel_Loader.coordSys(66).transform.translation  TranslationCartesianOffsetUnits=m  TranslationStandardAxis=+Z  TranslationStandardOffset=0  TranslationStandardOffsetUnits=m  TranslationROffset=0  TranslationROffsetUnits=m  TranslationThetaOffset=0  TranslationThetaOffsetUnits=deg  TranslationZOffset=0  TranslationZOffsetUnits=m
  RT_FrontFrame_Axle_Weld : sm_lib/Frames and Transforms/Rigid Transform  RotationMethod=RotationMatrix  FollAlignAxisA=+X  BaseAlignAxisA=+Y  FollAlignAxisB=+Y  BaseAlignAxisB=+Z  RotationStandardAxis=+Z  RotationAngle=0.0  RotationAngleUnits=deg  RotationArbitraryAxis=[0 0 1]  RotationSequenceAxes=FollowerAxes  RotationSequence=XYX  RotationSequenceAngles=[0 0 0]  RotationSequenceAnglesUnits=deg  RotationMatrix=[1 0 0; 0 1 0; 0 0 1]  Quaternion=[1 0 0 0]  TranslationMethod=Cartesian  TranslationCartesianOffset=[0 0 0]  TranslationCartesianOffsetUnits=m  TranslationStandardAxis=+Z  TranslationStandardOffset=0  TranslationStandardOffsetUnits=m  TranslationROffset=0  TranslationROffsetUnits=m  TranslationThetaOffset=0  TranslationThetaOffsetUnits=deg  TranslationZOffset=0  TranslationZOffsetUnits=m
  HFL : PMIOPort  Side=Left
  Frame : PMIOPort  Port=2  Side=Right
  HFP : PMIOPort  Port=3  Side=Left
  HFR : PMIOPort  Port=4  Side=Left
  connections:
  RT_FrontAxle_LFFDRing_Weld/RConn1 -- HFL/RConn1
  RT_FrontAxle_RFFDRing_Weld/RConn1 -- HFR/RConn1
  RT_FrontAxle_FDPinion/RConn1 -- HFP/RConn1
  RT_FrontFrame_Axle_Weld/RConn1 -- Frame/RConn1
  Housing/RConn1 -- Bolts/RConn1 -- Bearing/RConn1 -- RT_FrontFrame_Axle_Weld/LConn1 -- RT_FrontAxle_FDPinion/LConn1 -- RT_FrontAxle_RFFDRing_Weld/LConn1 -- RT_FrontAxle_LFFDRing_Weld/LConn1

== system sm_wheel_loader_lib/Wheel Loader Vehicle/Driveline/Axle Housing Rear ==
  Bolts : sm_lib/Body Elements/File Solid  ExtGeomFileName=AxleR_Housing_Bolts.STEP  UnitType=FromFile  ExtGeomFileUnits=m  StepReaderType=HEX  ExportConvexHullGeometry=off  InertiaType=Custom  BasedOnType=DensityFromFile  Density=1000  DensityUnits=kg/m^3  Mass=Wheel_Loader.bodyGroups(37).subGroups(2).inertialProperties.mass  MassUnits=kg  CenterOfMass=Wheel_Loader.bodyGroups(37).subGroups(2).inertialProperties.centerOfMass  CenterOfMassUnits=m  MomentsOfInertia=Wheel_Loader.bodyGroups(37).subGroups(2).inertialProperties.momentsOfInertia  MomentsOfInertiaUnits=kg*m^2  ProductsOfInertia=Wheel_Loader.bodyGroups(37).subGroups(2).inertialProperties.productsOfInertia  ProductsOfInertiaUnits=kg*m^2  GraphicType=FromGeometry  MarkerShape=Sphere  MarkerSize=10  GraphicVisPropType=SimpleVisualProperties  GraphicDiffuseColor=Wheel_Loader.bodyGroups(37).subGroups(2).visualProperties.rgb  GraphicOpacity=ra_casing_opc  GraphicSpecularColor=[0.5 0.5 0.5 1.0]  GraphicAmbientColor=[0.15 0.15 0.15 1.0]  GraphicEmissiveColor=[0.0 0.0 0.0 1.0]  GraphicShininess=75  DoExposeReferenceFrame=on  SerializedFrames=<Frames/>
  Housing : sm_lib/Body Elements/File Solid  ExtGeomFileName=AxleR_Housing.STEP  UnitType=FromFile  ExtGeomFileUnits=m  StepReaderType=HEX  ExportConvexHullGeometry=off  InertiaType=Custom  BasedOnType=DensityFromFile  Density=1000  DensityUnits=kg/m^3  Mass=Wheel_Loader.bodyGroups(37).subGroups(1).inertialProperties.mass  MassUnits=kg  CenterOfMass=Wheel_Loader.bodyGroups(37).subGroups(1).inertialProperties.centerOfMass  CenterOfMassUnits=m  MomentsOfInertia=Wheel_Loader.bodyGroups(37).subGroups(1).inertialProperties.momentsOfInertia  MomentsOfInertiaUnits=kg*m^2  ProductsOfInertia=Wheel_Loader.bodyGroups(37).subGroups(1).inertialProperties.productsOfInertia  ProductsOfInertiaUnits=kg*m^2  GraphicType=FromGeometry  MarkerShape=Sphere  MarkerSize=10  GraphicVisPropType=SimpleVisualProperties  GraphicDiffuseColor=Wheel_Loader.bodyGroups(37).subGroups(1).visualProperties.rgb  GraphicOpacity=ra_casing_opc  GraphicSpecularColor=[0.5 0.5 0.5 1.0]  GraphicAmbientColor=[0.15 0.15 0.15 1.0]  GraphicEmissiveColor=[0.0 0.0 0.0 1.0]  GraphicShininess=75  DoExposeReferenceFrame=on  SerializedFrames=<Frames/>
  RT_RearAxle_GBHousing_Weld : sm_lib/Frames and Transforms/Rigid Transform  RotationMethod=RotationMatrix  FollAlignAxisA=+X  BaseAlignAxisA=+Y  FollAlignAxisB=+Y  BaseAlignAxisB=+Z  RotationStandardAxis=+Z  RotationAngle=0.0  RotationAngleUnits=deg  RotationArbitraryAxis=[0 0 1]  RotationSequenceAxes=FollowerAxes  RotationSequence=XYX  RotationSequenceAngles=[0 0 0]  RotationSequenceAnglesUnits=deg  RotationMatrix=Wheel_Loader.coordSys(56).transform.rotation  Quaternion=[1 0 0 0]  TranslationMethod=Cartesian  TranslationCartesianOffset=Wheel_Loader.coordSys(56).transform.translation  TranslationCartesianOffsetUnits=m  TranslationStandardAxis=+Z  TranslationStandardOffset=0  TranslationStandardOffsetUnits=m  TranslationROffset=0  TranslationROffsetUnits=m  TranslationThetaOffset=0  TranslationThetaOffsetUnits=deg  TranslationZOffset=0  TranslationZOffsetUnits=m
  RT_RearAxle_LRFDRing_Weld : sm_lib/Frames and Transforms/Rigid Transform  RotationMethod=RotationMatrix  FollAlignAxisA=+X  BaseAlignAxisA=+Y  FollAlignAxisB=+Y  BaseAlignAxisB=+Z  RotationStandardAxis=+Z  RotationAngle=0.0  RotationAngleUnits=deg  RotationArbitraryAxis=[0 0 1]  RotationSequenceAxes=FollowerAxes  RotationSequence=XYX  RotationSequenceAngles=[0 0 0]  RotationSequenceAnglesUnits=deg  RotationMatrix=Wheel_Loader.coordSys(62).transform.rotation  Quaternion=[1 0 0 0]  TranslationMethod=Cartesian  TranslationCartesianOffset=Wheel_Loader.coordSys(62).transform.translation  TranslationCartesianOffsetUnits=m  TranslationStandardAxis=+Z  TranslationStandardOffset=0  TranslationStandardOffsetUnits=m  TranslationROffset=0  TranslationROffsetUnits=m  TranslationThetaOffset=0  TranslationThetaOffsetUnits=deg  TranslationZOffset=0  TranslationZOffsetUnits=m
  RT_RearAxle_RRFDRing_Weld : sm_lib/Frames and Transforms/Rigid Transform  RotationMethod=RotationMatrix  FollAlignAxisA=+X  BaseAlignAxisA=+Y  FollAlignAxisB=+Y  BaseAlignAxisB=+Z  RotationStandardAxis=+Z  RotationAngle=0.0  RotationAngleUnits=deg  RotationArbitraryAxis=[0 0 1]  RotationSequenceAxes=FollowerAxes  RotationSequence=XYX  RotationSequenceAngles=[0 0 0]  RotationSequenceAnglesUnits=deg  RotationMatrix=Wheel_Loader.coordSys(58).transform.rotation  Quaternion=[1 0 0 0]  TranslationMethod=Cartesian  TranslationCartesianOffset=Wheel_Loader.coordSys(58).transform.translation  TranslationCartesianOffsetUnits=m  TranslationStandardAxis=+Z  TranslationStandardOffset=0  TranslationStandardOffsetUnits=m  TranslationROffset=0  TranslationROffsetUnits=m  TranslationThetaOffset=0  TranslationThetaOffsetUnits=deg  TranslationZOffset=0  TranslationZOffsetUnits=m
  RT_RearFrame_Axle_Weld : sm_lib/Frames and Transforms/Rigid Transform  RotationMethod=RotationMatrix  FollAlignAxisA=+X  BaseAlignAxisA=+Y  FollAlignAxisB=+Y  BaseAlignAxisB=+Z  RotationStandardAxis=+Z  RotationAngle=0.0  RotationAngleUnits=deg  RotationArbitraryAxis=[0 0 1]  RotationSequenceAxes=FollowerAxes  RotationSequence=XYX  RotationSequenceAngles=[0 0 0]  RotationSequenceAnglesUnits=deg  RotationMatrix=[1 0 0; 0 1 0; 0 0 1]  Quaternion=[1 0 0 0]  TranslationMethod=Cartesian  TranslationCartesianOffset=[0 0 0]  TranslationCartesianOffsetUnits=m  TranslationStandardAxis=+Z  TranslationStandardOffset=0  TranslationStandardOffsetUnits=m  TranslationROffset=0  TranslationROffsetUnits=m  TranslationThetaOffset=0  TranslationThetaOffsetUnits=deg  TranslationZOffset=0  TranslationZOffsetUnits=m
  Frame : PMIOPort  Side=Left
  HRL : PMIOPort  Port=2  Side=Right
  HRP : PMIOPort  Port=3  Side=Right
  HRR : PMIOPort  Port=4  Side=Right
  connections:
  RT_RearAxle_LRFDRing_Weld/RConn1 -- HRL/RConn1
  RT_RearAxle_RRFDRing_Weld/RConn1 -- HRR/RConn1
  RT_RearAxle_GBHousing_Weld/RConn1 -- HRP/RConn1
  RT_RearFrame_Axle_Weld/RConn1 -- Frame/RConn1
  RT_RearAxle_RRFDRing_Weld/LConn1 -- RT_RearAxle_LRFDRing_Weld/LConn1 -- Housing/RConn1 -- Bolts/RConn1 -- RT_RearFrame_Axle_Weld/LConn1 -- RT_RearAxle_GBHousing_Weld/LConn1

== system sm_wheel_loader_lib/Wheel Loader Vehicle/Driveline/Driveline ==
  Driveline 1D : Subsystem  VariantControl=Driveline_1D
      settings: PortSchema="{\"entries\":[{\"content\":{\"sides\":[{\"content\":{\"connectorIds\":[\"LConn1\",\"LConn2\",\"LConn3\"]},\"type\":\"ConnectorPlacement.EquallySpacedRectSide\",\"uuid\":\"b63b559c-62bd-445e-b7ec-d91a1cc2405e\"},{\"content\":{\"connectorIds\":[\"RConn1\",\"RConn2\",\"RConn3\"],\"side\":\"RIGHT\"},\"type\":\"ConnectorPlacement.EquallySpacedRectSide\",\"uuid\":\"032d5054-ea2a-4303-8f34-205eab6388de\"},{\"content\":{\"connectorIds\":[\"LConn4\",\"LConn5\",\"LConn6\"],\"side\":\"TOP\"},\"type\":\"ConnectorPlacement.EquallySpacedRectSide\",\"uuid\":\"d2f0756e-9d37-498a-a5f3-0e74497a6223\"},{\"content\":{\"connectorIds\":[\"RConn4\",\"RConn5\",\"RConn6\"],\"side\":\"BOTTOM\"},\"type\":\"ConnectorPlacement.EquallySpacedRectSide\",\"uuid\":\"6a60c5c4-76fc-4699-b9fc-b8ae6c8913a6\"}]},\"type\":\"ConnectorPlacement.EquallySpacedConnector\",\"uuid\":\"1dc94a05-d7e7-41ec-b5c7-4a84600f46a8\"}],\"packageUris\":[\"http://schema.mathworks.com/mf0/Connector/R2020b\"],\"version\":\"1.0\"}"
      mask Display: image('sm_wheel_loader_driveline1D_IMAGE.png')
  Driveline 3D : Subsystem  VariantControl=Driveline_3D  mask{popup_driveJointF=CV Joint, popup_driveJointR=CV Joint}
      mask prompts: popup_driveJointF "Driveshaft Joint (front)"; popup_driveJointR "Driveshaft Joint (rear)"
      settings: PortSchema="{\"entries\":[{\"content\":{\"sides\":[{\"content\":{\"connectorIds\":[\"LConn1\",\"LConn2\",\"LConn3\"]},\"type\":\"ConnectorPlacement.EquallySpacedRectSide\",\"uuid\":\"ac94f403-7500-4d3b-9e0f-075c8f20a849\"},{\"content\":{\"connectorIds\":[\"RConn1\",\"RConn2\",\"RConn3\"],\"side\":\"RIGHT\"},\"type\":\"ConnectorPlacement.EquallySpacedRectSide\",\"uuid\":\"0eb844aa-00af-4edc-a570-50ab4e6b66c2\"},{\"content\":{\"connectorIds\":[\"LConn4\",\"LConn5\",\"LConn6\"],\"side\":\"TOP\"},\"type\":\"ConnectorPlacement.EquallySpacedRectSide\",\"uuid\":\"abddfcb0-9899-4667-9404-ac15e4716921\"},{\"content\":{\"connectorIds\":[\"RConn4\",\"RConn5\",\"RConn6\"],\"side\":\"BOTTOM\"},\"type\":\"ConnectorPlacement.EquallySpacedRectSide\",\"uuid\":\"a33fa760-6818-409d-ace3-b40bc7e3acff\"}]},\"type\":\"ConnectorPlacement.EquallySpacedConnector\",\"uuid\":\"2bc03850-1261-46ce-b9b6-2dbda85e9fb0\"}],\"packageUris\":[\"http://schema.mathworks.com/mf0/Connector/R2020b\"],\"version\":\"1.0\"}"
      mask TypeOptions popup_driveJointF:
      | Driveshaft
      | Front/popup_driveJointF
      mask TypeOptions popup_driveJointR:
      | Driveshaft
      | Rear/popup_driveJointR
      mask Display: image('sm_wheel_loader_driveline3D_IMAGE.png')
  wRL : PMIOPort  Side=Left
  Tr1 : PMIOPort  Port=2  Side=Left
  wFL : PMIOPort  Port=3  Side=Left
  HRL : PMIOPort  Port=4  Side=Left
  HRP : PMIOPort  Port=5  Side=Left
  HRR : PMIOPort  Port=6  Side=Left
  wRR : PMIOPort  Port=7  Side=Right
  Tr : PMIOPort  Port=8  Side=Right
  wFR : PMIOPort  Port=9  Side=Right
  HFL : PMIOPort  Port=10  Side=Right
  HFP : PMIOPort  Port=11  Side=Right
  HFR : PMIOPort  Port=12  Side=Right

== system sm_wheel_loader_lib/Wheel Loader Vehicle/Driveline/Wheel FL ==
  Hub : Subsystem  Tag=B230D770-3EF4-C446-A53F-6306E8DE466B
  Tire : Subsystem  Tag=1B5B75A7-7B5C-4849-8411-0061864F750D
  C : PMIOPort  Side=Left
  S : PMIOPort  Port=2  Side=Right
  connections:
  S/RConn1 -- Hub/LConn1
  Tire/LConn1 -- Hub/RConn1
  C/RConn1 -- Tire/RConn1

== system sm_wheel_loader_lib/Wheel Loader Vehicle/Driveline/Wheel FR ==
  Hub : Subsystem  Tag=5DF5B1C3-69E9-F644-9747-64BA6A51FD34
  Tire : Subsystem  Tag=2A7E39F9-3B28-3A4E-B0C7-8D7EA453C230
  S : PMIOPort  Side=Left
  C : PMIOPort  Port=2  Side=Right
  connections:
  S/RConn1 -- Hub/LConn1
  C/RConn1 -- Tire/RConn1
  Tire/LConn1 -- Hub/RConn1
